simulink model "sf_moore_vending_machine"  (R2025b)
settings: Solver=FixedStepDiscrete  StartTime=0.0  StopTime=200  FixedStep=1  RelTol=1e-3  EnableMultiTasking=on
settings Model: Creator=The MathWorks, Inc.  LastModifiedBy=The MathWorks, Inc.
settings SolverCC: AlgebraicLoopSolver=TrustRegion
settings DataIOCC: LimitDataPoints=on  SaveFormat=Array  ReturnWorkspaceOutputs=off  SignalLoggingName=sigsOut
settings OptimizationCC: ReuseModelBlockBuffer=off  ExpressionDepthLimit=2147483647.0  InitFltsAndDblsToZero=on  LifeSpan=inf
settings DebuggingCC: SaveWithParameterizedLinksMsg=none  UnderspecifiedInitializationDetection=Classic  MergeDetectMultiDrivingBlocksExec=none  SignalResolutionControl=TryResolveAllWithWarning  MultiTaskDSMMsg=warning  MultiTaskCondExecSysMsg=none  SigSpecEnsureSampleTimeMsg=none  FcnCallInpInsideContextMsg=warning  UnconnectedInputMsg=warning  UnconnectedOutputMsg=warning  UnconnectedLineMsg=warning  StateNameClashWarn=warning  SFUnexpectedBacktrackingDiag=warning  SFNoUnconditionalDefaultTransitionDiag=warning  SFExecutionAtInitializationDiag=none  ArithmeticOperatorsInVariantConditions=warning
settings HardwareCC: ProdBitPerPointer=32.0  ProdBitPerSizeT=32.0  ProdBitPerPtrDiffT=32.0  ProdLargestAtomicFloat=None  ProdIntDivRoundTo=Undefined  ProdEndianess=Unspecified  ProdWordSize=32.0  ProdHWDeviceType=32-bit Generic  TargetUnknown=on
settings ModelReferenceCC: EnableRefExpFcnMdlSchedulingChecks=on  PropagateSignalLabelsOutOfModel=off
settings SFSimCC: SimUseLocalCustomCode=off  CustomCodeUndefinedFunction=UseInterfaceOnly
settings RTWCC: RTWUseLocalCustomCode=off  GPUComputeCapability=3.5
settings CodeAppCC: StateflowObjectComments=on
settings GRTTargetCC: TargetFcnLib=ansi_tfl_tmw.mat  TargetLangStandard=C89/C90 (ANSI)  CombineOutputUpdateFcns=off  GRTInterface=on
settings ConfigComp: CovMetricSettings=dw  CovSaveCumulativeToWorkspaceVar=on  CovSaveSingleToWorkspaceVar=on  CovExternalEMLEnable=off

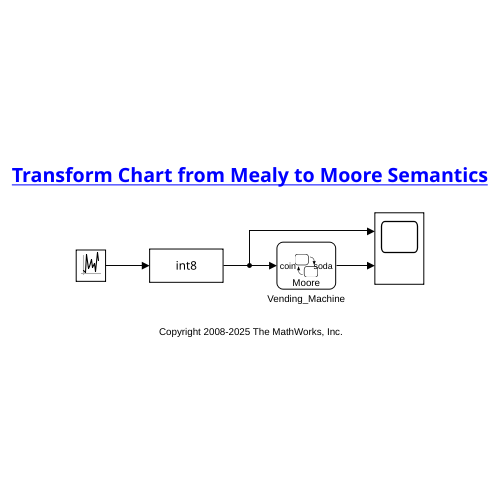
[thumbnail: Simulink's stored preview of the top-level diagram]
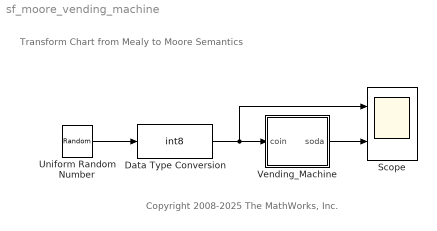
== system sf_moore_vending_machine ==
  note: Copyright 2008-2025 The MathWorks, Inc.
  note: Transform Chart from Mealy to Moore Semantics
  Data Type Conversion : DataTypeConversion  OutDataTypeStr=int8  RndMeth=Nearest
  Scope : Scope  NumInputPorts=2
      settings: ActiveDisplayYMinimum=-1  ActiveDisplayYMaximum=2
  Uniform Random Number : UniformRandomNumber  Minimum=0  Maximum=2  SampleTime=10
  Vending_Machine : Stateflow chart  TreatAsAtomicUnit=on
  wires:
  Uniform Random Number/1 -> Data Type Conversion/1
  Vending_Machine/1(soda) -> Scope/2
  Data Type Conversion/1 -> Vending_Machine/1(coin), Scope/1

== stateflow chart sf_moore_vending_machine/Vending_Machine ==
  settings: stateMachineType=MOORE_MACHINE  executeAtInitialization=1  initializeOutput=1
  state got_0
    soda = 0
  state got_nickel
    soda = 0
  state got_dime_dime
    soda = 1
  state got_dime
    soda = 0
  state got_dime_nickel
    soda = 1
  (default) -> got_0
  got_0 -> got_nickel [order 1] : [coin==1]
  got_dime_nickel -> got_0 [order 3]
  got_nickel -> got_dime [order 1] : [coin==1]
  got_0 -> got_dime [order 2] : [coin==2]
  got_dime_dime -> got_nickel [order 3]
  got_dime_nickel -> got_nickel [order 1] : [coin==1]
  got_nickel -> got_dime_nickel [order 2] : [coin==2]
  got_dime -> got_dime_dime [order 2] : [coin==2]
  got_dime_dime -> got_dime [order 1] : [coin==1]
  got_dime_dime -> got_dime_nickel [order 2] : [coin==2]
  got_dime_nickel -> got_dime [order 2] : [coin==2]
  got_dime -> got_dime_nickel [order 1] : [coin==1]
  data: coin input int8; soda output boolean
